simulink model "sf_ladder_logic_scheduler"  (R2025b)
settings: Solver=FixedStepDiscrete  StartTime=0.0  StopTime=10  RelTol=1e-3  EnableMultiTasking=on
model workspace (MAT data in the model file):
  deltat = 0.001
settings Model: Creator=The MathWorks, Inc.  LastModifiedBy=The MathWorks, Inc.
settings SolverCC: AlgebraicLoopSolver=TrustRegion  InsertRTBMode=Auto
settings DataIOCC: SaveFormat=Array  ReturnWorkspaceOutputs=off
settings OptimizationCC: ReuseModelBlockBuffer=off  ExpressionDepthLimit=2147483647.0  InitFltsAndDblsToZero=on  LifeSpan=inf
settings DebuggingCC: SaveWithParameterizedLinksMsg=none  UnderspecifiedInitializationDetection=Classic  MergeDetectMultiDrivingBlocksExec=none  SignalResolutionControl=TryResolveAllWithWarning  SolverPrmCheckMsg=warning  InheritedTsInSrcMsg=none  MultiTaskDSMMsg=warning  MultiTaskCondExecSysMsg=none  FcnCallInpInsideContextMsg=warning  UnconnectedInputMsg=warning  UnconnectedOutputMsg=warning  UnconnectedLineMsg=warning  StateNameClashWarn=warning  SFUnexpectedBacktrackingDiag=warning  SFNoUnconditionalDefaultTransitionDiag=warning  SFExecutionAtInitializationDiag=none  ArithmeticOperatorsInVariantConditions=warning
settings HardwareCC: ProdBitPerPointer=32.0  ProdBitPerSizeT=32.0  ProdBitPerPtrDiffT=32.0  ProdLargestAtomicFloat=None  ProdIntDivRoundTo=Undefined  ProdEndianess=Unspecified  ProdWordSize=32.0  ProdHWDeviceType=32-bit Generic
settings ModelReferenceCC: EnableRefExpFcnMdlSchedulingChecks=on  PropagateSignalLabelsOutOfModel=off
settings SFSimCC: SFSimEcho=off  SimUseLocalCustomCode=off  SimParseCustomCode=off
settings RTWCC: RTWUseLocalCustomCode=off  GPUComputeCapability=3.5
settings CodeAppCC: StateflowObjectComments=on
settings GRTTargetCC: TargetFcnLib=ansi_tfl_tmw.mat  TargetLangStandard=C89/C90 (ANSI)  CombineOutputUpdateFcns=off  GRTInterface=on
settings ConfigComp: CovMetricSettings=dw  CovSaveCumulativeToWorkspaceVar=on  CovSaveSingleToWorkspaceVar=on  CovExternalEMLEnable=off  CovSFcnEnable=off

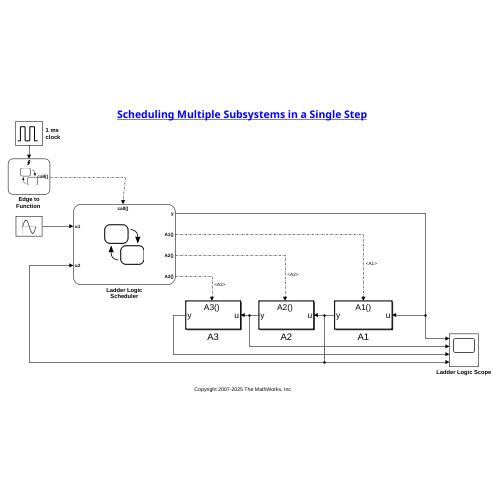
[thumbnail: Simulink's stored preview of the top-level diagram]
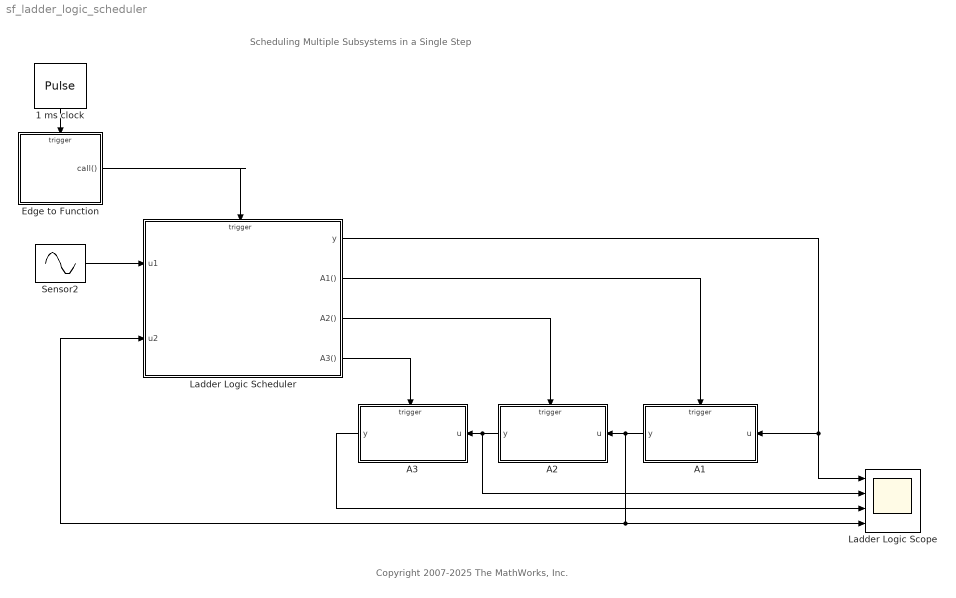
== system sf_ladder_logic_scheduler ==
  note: Copyright 2007-2025 The MathWorks, Inc.
  note: Scheduling Multiple Subsystems in a Single Step
  1 ms clock : DiscretePulseGenerator  PulseType=Time based  Period=0.001  PulseWidth=10
  A1 : Subsystem  TreatAsAtomicUnit=on
  A2 : Subsystem  TreatAsAtomicUnit=on
  A3 : Subsystem  TreatAsAtomicUnit=on
  "Edge to Function " : Stateflow chart  TreatAsAtomicUnit=on
  Ladder Logic Scheduler : Stateflow chart  TreatAsAtomicUnit=on
  Ladder Logic Scope : Scope  NumInputPorts=4
      settings: TimeSpan=0.5  Title=Output from Chart  ActiveDisplayYMinimum=-1.49985  ActiveDisplayYMaximum=3.49998
  Sensor2 : Sin  Frequency=40  Phase=-pi/8
  wires:
  Ladder Logic Scheduler/2(A1()) -> A1/Trigger
  Ladder Logic Scheduler/3(A2()) -> A2/Trigger
  A1/1(y) -> Ladder Logic Scheduler/2(u2), Ladder Logic Scope/4, A2/1(u)
  Ladder Logic Scheduler/1(y) -> Ladder Logic Scope/1, A1/1(u)
  Ladder Logic Scheduler/4(A3()) -> A3/Trigger
  1 ms clock/1 -> "Edge to Function "/Trigger
  Sensor2/1 -> Ladder Logic Scheduler/1(u1)
  "Edge to Function "/1(call()) -> Ladder Logic Scheduler/Trigger
  A2/1(y) -> Ladder Logic Scope/2, A3/1(u)
  A3/1(y) -> Ladder Logic Scope/3

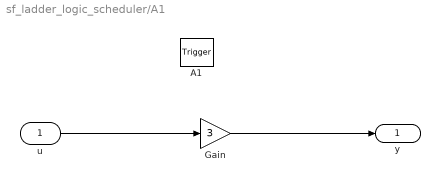
== system sf_ladder_logic_scheduler/A1 ==
  u : Inport
  A1 : TriggerPort  TriggerType=function-call  VariantControl=(inherit)
  Gain : Gain  Gain=3
  y : Outport  VectorParamsAs1DForOutWhenUnconnected=off
  wires:
  u/1 -> Gain/1
  Gain/1 -> y/1

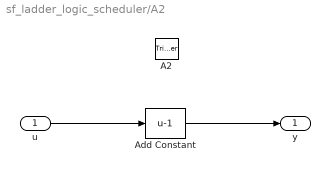
== system sf_ladder_logic_scheduler/A2 ==
  u : Inport
  A2 : TriggerPort  TriggerType=function-call  VariantControl=(inherit)
  Add Constant : Bias  Bias=-1  SaturateOnIntegerOverflow=off
  y : Outport  InitialOutput=0  VectorParamsAs1DForOutWhenUnconnected=off
  wires:
  u/1 -> Add Constant/1
  Add Constant/1 -> y/1

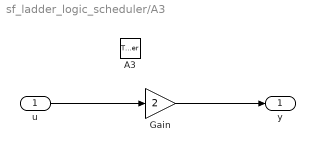
== system sf_ladder_logic_scheduler/A3 ==
  u : Inport
  A3 : TriggerPort  TriggerType=function-call  VariantControl=(inherit)
  Gain : Gain  Gain=2
  y : Outport  VectorParamsAs1DForOutWhenUnconnected=off
  wires:
  u/1 -> Gain/1
  Gain/1 -> y/1

== stateflow chart sf_ladder_logic_scheduler/Ladder Logic Scheduler ==
  settings: executeAtInitialization=1
  (default) -> (junction 12) : {y=u1;}
  (junction 12) -> (junction 13) [order 1] : [u1>0]
  (junction 12) -> (junction 14) [order 2]
  (junction 13) -> (junction 14) : {send(A1)}
  (junction 14) -> (junction 15) [order 1] : [u2>1]
  (junction 14) -> (junction 16) [order 2]
  (junction 15) -> (junction 16) : {send(A2)}
  (junction 16) -> (junction 17) [order 1] : [u2<2]
  (junction 16) -> (junction 18) [order 2]
  (junction 17) -> (junction 18) : {send(A3)}
  data: y output double; u1 input; u2 input
  events: A1 output FUNCTION_CALL_EVENT; A2 output FUNCTION_CALL_EVENT; A3 output FUNCTION_CALL_EVENT; call input FUNCTION_CALL_EVENT

== stateflow chart sf_ladder_logic_scheduler/Edge to Function  ==
  settings: executeAtInitialization=1
  (default) -> (junction 2) : {call;}
  events: edge input RISING_EDGE_EVENT; call output FUNCTION_CALL_EVENT
